simulink model "fft_test"  (Simulink 7.4)
settings: Solver=VariableStepDiscrete  StartTime=0.0  StopTime=500  RelTol=1e-3
libraries: xbsIndex_r4 x1178, casper_library_misc x68, casper_library_delays x13, casper_library_reorder x4, casper_library_ffts_twiddle x2
(part 1 of 11)
settings Model: Creator=User  LastModifiedBy=wjm
settings OptimizationCC: InitFltsAndDblsToZero=on
settings DebuggingCC: SaveWithDisabledLinksMsg=none  SaveWithParameterizedLinksMsg=none

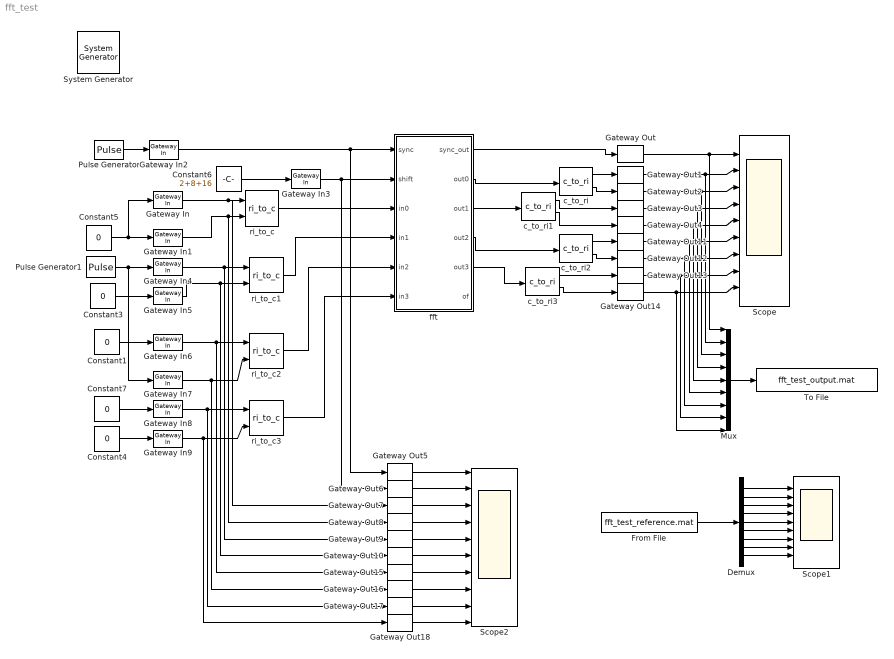
== system fft_test ==
  " System Generator" : xbsIndex_r4/ System Generator  Tag=genX  SystemSampleTime=-1  xilinxfamily=virtex5  part=xc5vsx95t  speed=-1  package=ff1136  synthesis_tool=XST  clock_wrapper=Clock Enables  directory=./netlist  testbench=off  simulink_period=1  sysclk_period=100  dcm_input_clock_period=100  incr_netlist=off  trim_vbits=Everywhere in SubSystem  dbl_ovrd=According to Block Masks  core_generation=According to Block Masks  run_coregen=off  deprecated_control=off  eval_field=0  block_type=sysgen
      settings: block_version=10.1.1
  Constant{1,3..5,7} (5 alike) : Constant  Value=0  OutDataType=sfix(16)  OutScaling=2^0
  Constant6 : Constant  Value=2+8+16  OutDataType=sfix(16)  OutScaling=2^0
  Demux : Demux  Outputs=9
  From File : FromFile  FileName=fft_test_reference.mat  SampleTime=1
  Gateway In{,1,4..9} (8 alike) : xbsIndex_r4/Gateway In  arith_type="Signed  (2's comp)"  n_bits=8  bin_pt=7  quantization=Truncate  overflow=Wrap  period=1  dbl_ovrd=off  timing_constraint=None  locs_specified=off  LOCs={}  hdl_port=on  block_type=gatewayin
      settings: infoedit="Gateway in block.  Converts inputs of type Simulink integer, double and fixed point to  Xilinx fixed point type.<P><P>Hardware notes:  In hardware these blocks become top level input ports."  block_version=10.1.1
  Gateway In2 : xbsIndex_r4/Gateway In  arith_type=Boolean  n_bits=18  bin_pt=17  quantization=Truncate  overflow=Wrap  period=1  dbl_ovrd=off  timing_constraint=None  locs_specified=off  LOCs={}  hdl_port=on  block_type=gatewayin
      settings: infoedit="Gateway in block.  Converts inputs of type Simulink integer, double and fixed point to  Xilinx fixed point type.<P><P>Hardware notes:  In hardware these blocks become top level input ports."  block_version=10.1.1
  Gateway In3 : xbsIndex_r4/Gateway In  arith_type=Unsigned  n_bits=11  bin_pt=0  quantization=Truncate  overflow=Wrap  period=1  dbl_ovrd=off  timing_constraint=None  locs_specified=off  LOCs={}  hdl_port=on  block_type=gatewayin
      settings: infoedit="Gateway in block.  Converts inputs of type Simulink integer, double and fixed point to  Xilinx fixed point type.<P><P>Hardware notes:  In hardware these blocks become top level input ports."  block_version=10.1.1
  Gateway Out{,1..18} (19 alike) : xbsIndex_r4/Gateway Out  hdl_port=on  timing_constraint=None  locs_specified=off  LOCs={}  block_type=gatewayout
      settings: infoedit="Gateway out block.  Converts Xilinx fixed point inputs into ouputs of type Simulink integer, double, or fixed point.<P><P>Hardware notes:  In hardware these blocks become top level output ports or are discarded, depending on how they are configured."  block_version=10.1.1
  Mux : Mux  Inputs=9
  Pulse Generator : DiscretePulseGenerator  Amplitude=1  Period=2^7  PulseWidth=1  PhaseDelay=11  SampleTime=1
  Pulse Generator1 : DiscretePulseGenerator  Amplitude=0.5  Period=2^4  PulseWidth=1  PhaseDelay=12  SampleTime=1
  Scope : Scope  NumInputPorts=9
      settings: YMin=-1~0~0~-5~-5~-5~-5~-5~-5  YMax=2~1~1~5~5~5~5~5~5
  Scope1 : Scope  NumInputPorts=9
      settings: YMin=-1~0~0~-5~-5~-5~-5~-5~-5  YMax=2~1~1~5~5~5~5~5~5
  Scope2 : Scope  NumInputPorts=10
      settings: YMin=-1~0~0~-5~-5~-5~-5~-5~-5~-5  YMax=2~1~1~5~5~5~5~5~5~5  SaveName=ScopeData2
  To File : ToFile  Filename=fft_test_output.mat  MatrixName=output
  c_to_ri{,1..3} (4 alike) : casper_library_misc/c_to_ri  SystemSampleTime=-1  n_bits=8  bin_pt=7
      settings: AttributesFormatString=8_7 r/i
  fft : Subsystem  AncestorBlock=casper_library_ffts/fft  mask(fft){FFTSize=6, input_bit_width=8, coeff_bit_width=8, n_inputs=2, quantization=Round  (unbiased: +/- Inf), overflow=Saturate, add_latency=2, mult_latency=3, bram_latency=1, conv_latency=2, arch=Virtex5, opt_target=multipliers, coeffs_bit_limit=8, delays_bit_limit=9, specify_mult=on, mult_spec=getfield( getfield( get_param( gcb,'UserData' ), 'parameters'),'mult_spec'), dsp48_adders=on}
      mask prompts: FFTSize "Size of FFT: (2^?)"; input_bit_width "Input/Output Bit Width"; coeff_bit_width "Coefficient Bit Width"; n_inputs "Number of Simultaneous Inputs: (2^?)"; quantization "Quantization Behavior"; overflow "Overflow Behavior"; add_latency "Add Latency"; mult_latency "Mult Latency"; bram_latency "BRAM Latency"; conv_latency "Convert latency"; arch "Architecture"; opt_target "Use less"; coeffs_bit_limit "Number bits above which to store stage's coefficients in BRAM (2^? bits)"; delays_bit_limit "Number bits above which to store stage's delays in BRAM (2^? bits)"; specify_mult "Specify multiplier use (behavioral HDL if not specified)"; mult_spec "Multiplier specification (0=core, 1=embedded, 2=behavioural) (left=1st stage)"; dsp48_adders "DSP48 adders in butterfly"
      mask init:
      | fft_init(gcb,...
      |     'FFTSize', FFTSize, ...
      |     'input_bit_width', input_bit_width, ...
      |     'coeff_bit_width', coeff_bit_width, ...
      |     'n_inputs', n_inputs, ...
      |     'quantization', quantization, ...
      |     'overflow', overflow, ...
      |     'add_latency', add_latency, ...
      |     'mult_latency', mult_latency, ...
      |     'bram_latency', bram_latency, ...
      |     'conv_latency', conv_latency, ...
      |     'arch', arch, ...
      |     'opt_target', opt_target, ...
      |     'coeffs_bit_limit', coeffs_bit_limit, ...
      |     'delays_bit_limit', delays_bit_limit, ...
      |     'specify_mult', specify_mult, ...
      |     'mult_spec', mult_spec, ...
      |     'dsp48_adders', dsp48_adders);
      settings: AttributesFormatString=|
      | 6 stages
      | (8,8)
      | Round  (unbiased: +/- Inf)
      | Saturate
      mask Help: eval('xlWeb(''http://casper.berkeley.edu/wiki/Fft'')')
      mask StyleString: edit,edit,edit,edit,popup(Truncate|Round  (unbiased: +/- Inf)|Round  (unbiased: Even Values)),popup(Wrap|Saturate|Error),edit,edit,edit,edit,popup(Virtex2Pro|Virtex5),popup(logic|multipliers),edit,edit,checkbox,edit,checkbox
      mask CallbackString:
      | % fft_size = eval(get_param(gcb, 'FFTSize'));
      | % old_vec = eval(get_param(gcb, 'mult_spec'));
      | 
      | % vec = 2.*ones(1,fft_size);
      | % old_size = length(old_vec);
      | 
      | % if(old_size <= fft_size), size = old_size;
      | % else, size = fft_size;
      | % end
      | 
      | % for n = 1:size, vec(n) = old_vec(n); end
      | % set_param(gcb, 'mult_spec', mat2str(vec));||||||||||fft_callback_arch(gcb);||||specify_mult = get_param(gcb,'specify_mult');
      | visibs = get_param(gcb, 'MaskVisibilities');
      | if( strcmp(specify_mult,'off')), visibs{16} = 'off';
      | else visibs{16} = 'on';
      | end
      | set_param(gcb, 'MaskVisibilities', visibs);
      | 
      | |% vec = eval( get_param(gcb, 'mult_spec'));
      | % vec_size = length(vec);
      | % fft_size = eval( get_param(gcb, 'FFTSize'));
      | % new_vec = 2.*ones(1, fft_size);
      | 
      | % if(vec_size <= fft_size), size = vec_size;
      | % else size = fft_size;
      | % end
      | 
      | % for n=1:size,
      | %    new_vec(n) = vec(n);
      | % end
      | % set_param(gcb, 'mult_spec', mat2str(new_vec));|fft_callback_dsp48_adders(gcb);
  ri_to_c{,1..3} (4 alike) : casper_library_misc/ri_to_c  SystemSampleTime=-1
  wires:
  Pulse Generator/1 -> Gateway In2/1
  Gateway In2/1 -> Gateway Out5/1, fft/1(sync)
  Gateway In3/1 -> Gateway Out6/1, fft/2(shift)
  fft/1(sync_out) -> Gateway Out/1
  fft/2(out0) -> c_to_ri/1
  c_to_ri/1 -> Gateway Out1/1
  c_to_ri/2 -> Gateway Out2/1
  c_to_ri1/2 -> Gateway Out4/1
  fft/3(out1) -> c_to_ri1/1
  c_to_ri1/1 -> Gateway Out3/1
  Gateway Out/1 -> Scope/1, Mux/1
  Gateway In/1 -> ri_to_c/1, Gateway Out7/1
  Gateway In1/1 -> ri_to_c/2, Gateway Out8/1
  Gateway In4/1 -> ri_to_c1/1, Gateway Out9/1
  Gateway In5/1 -> ri_to_c1/2, Gateway Out10/1
  Gateway Out1/1 -> Scope/2, Mux/2
  Gateway Out2/1 -> Scope/3, Mux/3
  Mux/1 -> To File/1
  Demux/1 -> Scope1/1
  Demux/2 -> Scope1/2
  Demux/3 -> Scope1/3
  Demux/4 -> Scope1/4
  Demux/5 -> Scope1/5
  Gateway Out5/1 -> Scope2/1
  Gateway Out6/1 -> Scope2/2
  Gateway Out7/1 -> Scope2/3
  Gateway Out8/1 -> Scope2/4
  Gateway Out9/1 -> Scope2/5
  Gateway Out10/1 -> Scope2/6
  Constant4/1 -> Gateway In9/1
  Gateway In6/1 -> ri_to_c2/1, Gateway Out15/1
  Gateway In7/1 -> ri_to_c2/2, Gateway Out16/1
  Gateway In8/1 -> ri_to_c3/1, Gateway Out17/1
  Gateway In9/1 -> ri_to_c3/2, Gateway Out18/1
  ri_to_c/1 -> fft/3(in0)
  ri_to_c1/1 -> fft/4(in1)
  ri_to_c2/1 -> fft/5(in2)
  ri_to_c3/1 -> fft/6(in3)
  c_to_ri2/1 -> Gateway Out11/1
  c_to_ri2/2 -> Gateway Out12/1
  c_to_ri3/1 -> Gateway Out13/1
  c_to_ri3/2 -> Gateway Out14/1
  Gateway Out3/1 -> Scope/4, Mux/4
  Gateway Out4/1 -> Scope/5, Mux/5
  Gateway Out11/1 -> Scope/6, Mux/6
  Gateway Out12/1 -> Scope/7, Mux/7
  Gateway Out13/1 -> Scope/8, Mux/8
  Gateway Out14/1 -> Scope/9, Mux/9
  Gateway Out15/1 -> Scope2/7
  Gateway Out16/1 -> Scope2/8
  Gateway Out17/1 -> Scope2/9
  Gateway Out18/1 -> Scope2/10
  From File/1 -> Demux/1
  Demux/6 -> Scope1/6
  Demux/7 -> Scope1/7
  Demux/8 -> Scope1/8
  Demux/9 -> Scope1/9
  Constant3/1 -> Gateway In5/1
  Constant5/1 -> Gateway In1/1, Gateway In/1
  Constant6/1 -> Gateway In3/1
  Constant1/1 -> Gateway In6/1
  Constant7/1 -> Gateway In8/1
  Pulse Generator1/1 -> Gateway In4/1, Gateway In7/1
  fft/4(out2) -> c_to_ri2/1
  fft/5(out3) -> c_to_ri3/1

== system fft_test/fft ==
  sync : Inport
  shift : Inport  Port=2
  in0 : Inport  Port=3
  in1 : Inport  Port=4
  in2 : Inport  Port=5
  in3 : Inport  Port=6
  fft_biplex0 : Subsystem  AncestorBlock=casper_library_ffts/fft_biplex  mask(fft_biplex){FFTSize=4, input_bit_width=8, coeff_bit_width=8, quantization=Round  (unbiased: +/- Inf), overflow=Saturate, add_latency=2, mult_latency=3, bram_latency=1, conv_latency=2, arch=Virtex5, opt_target=multipliers, coeffs_bit_limit=8, delays_bit_limit=9, specify_mult=on, mult_spec=getfield( getfield( get_param( gcb,'UserData' ), 'parameters'),'mult_spec'), dsp48_adders=on}
      mask prompts: FFTSize "Size of FFT: (2^? pnts)"; input_bit_width "Input/Output Bit Width"; coeff_bit_width "Coefficient Bit Width"; quantization "Quantization Behavior"; overflow "Overflow Behavior"; add_latency "Add Latency"; mult_latency "Mult Latency"; bram_latency "BRAM Latency"; conv_latency "Convert latency"; arch "Architecture"; opt_target "Use less"; coeffs_bit_limit "Number bits above which to store stage's coefficients in BRAM (2^? bits)"; delays_bit_limit "Number bits above which to implent stage's delays in BRAM (2^? bits)"; specify_mult "Specify multiplier use (behavioral HDL if not specified)"; mult_spec "Multiplier specification (0=core, 1=embedded, 2=behavioural) (left=1st stage)"; dsp48_adders "Use DSP48s for adders"
      mask init:
      | fft_biplex_init(gcb,...
      |     'FFTSize', FFTSize,...
      |     'input_bit_width', input_bit_width,...
      |     'coeff_bit_width', coeff_bit_width,...
      |     'quantization', quantization,...
      |     'overflow', overflow,...
      |     'add_latency', add_latency,...
      |     'mult_latency', mult_latency,...
      |     'bram_latency', bram_latency,...
      |     'conv_latency', conv_latency, ...
      |     'arch', arch, ...
      |     'opt_target', opt_target, ...
      |     'coeffs_bit_limit', coeffs_bit_limit, ...
      |     'delays_bit_limit', delays_bit_limit, ...
      |     'specify_mult', specify_mult,...
      |     'mult_spec', mult_spec, ...
      |     'dsp48_adders', dsp48_adders);
      settings: AttributesFormatString=|
      | 4 stages
      | Virtex5
      mask StyleString: edit,edit,edit,popup(Truncate|Round  (unbiased: +/- Inf)|Round  (unbiased: Even Values)),popup(Wrap|Saturate|Error),edit,edit,edit,edit,popup(Virtex2Pro|Virtex5),popup(logic|multipliers),edit,edit,checkbox,edit,checkbox
      mask CallbackString:
      | % fft_size = eval(get_param(gcb, 'FFTSize'));
      | % old_vec = eval(get_param(gcb, 'mult_spec'));
      | 
      | % vec = 2.*ones(1,fft_size);
      | % old_size = length(old_vec);
      | 
      | % if(old_size <= fft_size),
      | %    size = old_size;
      | % else,
      | %     size = fft_size;
      | % end
      | 
      | % for n = 1:size, vec(n) = old_vec(n); end
      | % set_param(gcb, 'mult_spec', mat2str(vec));|||||||||fft_callback_arch(gcb);||||specify_mult = get_param(gcb,'specify_mult');
      | visibs = get_param(gcb, 'MaskVisibilities');
      | 
      | if( strcmp(specify_mult,'off')), visibs{15} = 'off';
      | else, visibs{15} = 'on';
      | end
      | set_param(gcb, 'MaskVisibilities', visibs);
      | |% vec = eval( get_param(gcb, 'mult_spec'));
      | % vec_size = length(vec);
      | % fft_size = eval( get_param(gcb, 'FFTSize'));
      | % new_vec = 2.*ones(1, fft_size);
      | 
      | % if(vec_size <= fft_size), size = vec_size;
      | % else size = fft_size;
      | % end
      | 
      | % for n=1:size
      | %     new_vec(n) = vec(n);
      | % end
      | % set_param(gcb, 'mult_spec', mat2str(new_vec));|fft_callback_dsp48_adders(gcb);
  fft_biplex1 : Subsystem  AncestorBlock=casper_library_ffts/fft_biplex  mask(fft_biplex){FFTSize=4, input_bit_width=8, coeff_bit_width=8, quantization=Round  (unbiased: +/- Inf), overflow=Saturate, add_latency=2, mult_latency=3, bram_latency=1, conv_latency=2, arch=Virtex5, opt_target=multipliers, coeffs_bit_limit=8, delays_bit_limit=9, specify_mult=on, mult_spec=getfield( getfield( get_param( gcb,'UserData' ), 'parameters'),'mult_spec'), dsp48_adders=on}
      mask prompts: FFTSize "Size of FFT: (2^? pnts)"; input_bit_width "Input/Output Bit Width"; coeff_bit_width "Coefficient Bit Width"; quantization "Quantization Behavior"; overflow "Overflow Behavior"; add_latency "Add Latency"; mult_latency "Mult Latency"; bram_latency "BRAM Latency"; conv_latency "Convert latency"; arch "Architecture"; opt_target "Use less"; coeffs_bit_limit "Number bits above which to store stage's coefficients in BRAM (2^? bits)"; delays_bit_limit "Number bits above which to implent stage's delays in BRAM (2^? bits)"; specify_mult "Specify multiplier use (behavioral HDL if not specified)"; mult_spec "Multiplier specification (0=core, 1=embedded, 2=behavioural) (left=1st stage)"; dsp48_adders "Use DSP48s for adders"
      mask init: same as fft_test/fft/fft_biplex0
      settings: AttributesFormatString=|
      | 4 stages
      | Virtex5
      mask StyleString: edit,edit,edit,popup(Truncate|Round  (unbiased: +/- Inf)|Round  (unbiased: Even Values)),popup(Wrap|Saturate|Error),edit,edit,edit,edit,popup(Virtex2Pro|Virtex5),popup(logic|multipliers),edit,edit,checkbox,edit,checkbox
      mask CallbackString:
      | % fft_size = eval(get_param(gcb, 'FFTSize'));
      | % old_vec = eval(get_param(gcb, 'mult_spec'));
      | 
      | % vec = 2.*ones(1,fft_size);
      | % old_size = length(old_vec);
      | 
      | % if(old_size <= fft_size),
      | %    size = old_size;
      | % else,
      | %     size = fft_size;
      | % end
      | 
      | % for n = 1:size, vec(n) = old_vec(n); end
      | % set_param(gcb, 'mult_spec', mat2str(vec));|||||||||fft_callback_arch(gcb);||||specify_mult = get_param(gcb,'specify_mult');
      | visibs = get_param(gcb, 'MaskVisibilities');
      | 
      | if( strcmp(specify_mult,'off')), visibs{15} = 'off';
      | else, visibs{15} = 'on';
      | end
      | set_param(gcb, 'MaskVisibilities', visibs);
      | |% vec = eval( get_param(gcb, 'mult_spec'));
      | % vec_size = length(vec);
      | % fft_size = eval( get_param(gcb, 'FFTSize'));
      | % new_vec = 2.*ones(1, fft_size);
      | 
      | % if(vec_size <= fft_size), size = vec_size;
      | % else size = fft_size;
      | % end
      | 
      | % for n=1:size
      | %     new_vec(n) = vec(n);
      | % end
      | % set_param(gcb, 'mult_spec', mat2str(new_vec));|fft_callback_dsp48_adders(gcb);
  fft_direct : Subsystem  AncestorBlock=casper_library_ffts/fft_direct  mask(fft_direct){FFTSize=2, input_bit_width=8, coeff_bit_width=8, add_latency=2, mult_latency=3, bram_latency=1, conv_latency=2, quantization=Round  (unbiased: +/- Inf), overflow=Saturate, map_tail=on, LargerFFTSize=6, StartStage=5, arch=Virtex5, opt_target=multipliers, coeffs_bit_limit=8, specify_mult=on, mult_spec=[1                                      2], dsp48_adders=on}
      mask prompts: FFTSize "Size of FFT: (2^?)"; input_bit_width "Input/Output Bit Width"; coeff_bit_width "Coefficient Bit Width"; add_latency "Add Latency"; mult_latency "Mult Latency"; bram_latency "BRAM Latency"; conv_latency "Convert latency"; quantization "Quantization Behavior"; overflow "Overflow Behavior"; map_tail "Map Tail of Larger FFT"; LargerFFTSize "Size of Larger FFT (2^?):"; StartStage "Start Stage of Map Tail:"; arch "Architecture"; opt_target "Use less"; coeffs_bit_limit "Number bits above which to store stage's coefficients in BRAM (2^? bits)"; specify_mult "Specify multiplier use (behavioural HDL if not specified)"; mult_spec "Multiplier specification (0=core, 1=behavioural HDL, 2=embedded) (left=1st stage)"; dsp48_adders "DSP48 adders in butterfly"
      mask help:
      | Implements an N-point FFT with the classic
      | butterfly structure with N inputs and N outputs
      mask init:
      | fft_direct_init(gcb,...
      |     'FFTSize', FFTSize, ...
      |     'input_bit_width', input_bit_width, ...
      |     'coeff_bit_width', coeff_bit_width, ...
      |     'add_latency', add_latency, ...
      |     'mult_latency', mult_latency, ...
      |     'bram_latency', bram_latency, ...
      |     'conv_latency', conv_latency, ...
      |     'quantization', quantization, ...
      |     'overflow', overflow, ...
      |     'map_tail', map_tail, ...
      |     'LargerFFTSize', LargerFFTSize, ...
      |     'StartStage', StartStage, ...
      |     'arch', arch, ...
      |     'opt_target', opt_target, ...
      |     'coeffs_bit_limit', coeffs_bit_limit, ...
      |     'specify_mult', specify_mult, ...
      |     'mult_spec', mult_spec, ...
      |     'dsp48_adders', dsp48_adders);
      settings: AttributesFormatString=|
      | Virtex5
      | stages [5  6] of 6
      | [8,8]
      | Round  (unbiased: +/- Inf)
      | Saturate
      mask StyleString: edit,edit,edit,edit,edit,edit,edit,popup(Truncate|Round  (unbiased: +/- Inf)|Round  (unbiased: Even Values)),popup(Wrap|Saturate|Error),checkbox,edit,edit,popup(Virtex2Pro|Virtex5),popup(logic|multipliers),edit,checkbox,edit,checkbox
      mask CallbackString:
      | % fft_size = eval(get_param(gcb, 'FFTSize'));
      | % old_vec = eval(get_param(gcb, 'mult_spec'));
      | 
      | % vec = 2.*ones(1,fft_size);
      | % old_size = length(old_vec);
      | 
      | % if(old_size <= fft_size),
      | %     size = old_size;
      | % else,
      | %     size = fft_size;
      | % end
      | 
      | % for n = 1:size, vec(n) = old_vec(n); end
      | % set_param(gcb, 'mult_spec', mat2str(vec));|||||||||map_tail = get_param(gcb,'map_tail');
      | visibs = get_param(gcb, 'MaskVisibilities');
      | if( strcmp(map_tail,'off')),
      |     visibs{11} = 'off';
      |     visibs{12} = 'off';
      | else,
      |     visibs{11} = 'on';
      |     visibs{12} = 'on';
      | end
      | set_param(gcb, 'MaskVisibilities', visibs);
      | |||fft_callback_arch(gcb);|||specify_mult = get_param(gcb,'specify_mult');
      | visibs = get_param(gcb, 'MaskVisibilities');
      | if( strcmp(specify_mult,'off')), visibs{17} = 'off';
      | else, visibs{17} = 'on';
      | end
      | set_param(gcb, 'MaskVisibilities', visibs);
      | |% vec = eval( get_param(gcb, 'mult_spec'));
      | % vec_size = length(vec);
      | % fft_size = eval( get_param(gcb, 'FFTSize'));
      | % new_vec = 2.*ones(1, fft_size);
      | 
      | % if(vec_size <= fft_size), size = vec_size;
      | % else size = fft_size;
      | % end
      | 
      | % for n=1:size
      | %     new_vec(n) = vec(n);
      | % end
      | % set_param(gcb, 'mult_spec', mat2str(new_vec));|fft_callback_dsp48_adders(gcb);
  fft_unscrambler : Subsystem  AncestorBlock=casper_library_ffts/fft_unscrambler  mask(fft_unscrambler){FFTSize=6, n_inputs=2, bram_latency=1}
      mask prompts: FFTSize "Size of FFT: (2^?)"; n_inputs "Number of Simultaneous Inputs: (2^?)"; bram_latency "BRAM Latency"
      mask init:
      | fft_unscrambler_init(gcb,...
      |     'FFTSize',FFTSize,... 
      |     'n_inputs', n_inputs,...
      |     'bram_latency', bram_latency);
      settings: AttributesFormatString=FFTSize=6, n_inputs=2
  of_or : xbsIndex_r4/Logical  logical_function=OR  inputs=3  en=off  latency=1  precision=Full  arith_type=Unsigned  n_bits=16  bin_pt=0  align_bp=on  dbl_ovrd=off  block_type=logical
      settings: block_version=11.4
  slice : xbsIndex_r4/Slice  nbits=2  boolean_output=off  mode=Lower Bit Location + Width  bit1=0  base1=MSB of Input  bit0=4  base0=LSB of Input  dbl_ovrd=off  block_type=slice
  sync_out : Outport
  out0 : Outport  Port=2
  out1 : Outport  Port=3
  out2 : Outport  Port=4
  out3 : Outport  Port=5
  of : Outport  Port=6
  wires:
  in0/1 -> fft_biplex0/1(pol1)
  in1/1 -> fft_biplex0/2(pol2)
  shift/1 -> fft_biplex0/4(shift), fft_biplex1/4(shift), slice/1
  sync/1 -> fft_biplex0/3(sync), fft_biplex1/3(sync)
  fft_biplex0/3(of) -> of_or/2
  in2/1 -> fft_biplex1/1(pol1)
  in3/1 -> fft_biplex1/2(pol2)
  fft_biplex1/3(of) -> of_or/3
  slice/1 -> fft_direct/2(shift)
  fft_biplex0/4(sync_out) -> fft_direct/1(sync)
  fft_biplex0/1(pol1_out) -> fft_direct/3(in0)
  fft_biplex0/2(pol2_out) -> fft_direct/4(in1)
  fft_biplex1/1(pol1_out) -> fft_direct/5(in2)
  fft_biplex1/2(pol2_out) -> fft_direct/6(in3)
  fft_direct/6(of) -> of_or/1
  of_or/1 -> of/1
  fft_direct/1(sync_out) -> fft_unscrambler/1(sync)
  fft_unscrambler/1(sync_out) -> sync_out/1
  fft_direct/2(out0) -> fft_unscrambler/2(In1)
  fft_unscrambler/2(Out1) -> out0/1
  fft_direct/3(out1) -> fft_unscrambler/3(In2)
  fft_unscrambler/3(Out2) -> out1/1
  fft_direct/4(out2) -> fft_unscrambler/4(In3)
  fft_unscrambler/4(Out3) -> out2/1
  fft_direct/5(out3) -> fft_unscrambler/5(In4)
  fft_unscrambler/5(Out4) -> out3/1

== system fft_test/fft/fft_biplex0 ==
  pol1 : Inport  OutDataType=sfix(16)  OutScaling=2^0
  pol2 : Inport  Port=2  OutDataType=sfix(16)  OutScaling=2^0
  sync : Inport  Port=3  OutDataType=sfix(16)  OutScaling=2^0
  shift : Inport  Port=4  OutDataType=sfix(16)  OutScaling=2^0
  biplex_core : Subsystem  AncestorBlock=casper_library_ffts/biplex_core  mask(biplex_core){FFTSize=4, input_bit_width=8, coeff_bit_width=8, quantization=Round  (unbiased: +/- Inf), overflow=Saturate, add_latency=2, mult_latency=3, bram_latency=1, conv_latency=2, arch=Virtex5, opt_target=multipliers, coeffs_bit_limit=8, delays_bit_limit=9, specify_mult=on, mult_spec=getfield( getfield( get_param( gcb,'UserData' ), 'parameters'),'mult_spec'), dsp48_adders=on}
      mask prompts: FFTSize "Size of FFT: (2^? pnts)"; input_bit_width "Input/Output Bit Width"; coeff_bit_width "Coefficient Bit Width"; quantization "Quantization Behavior"; overflow "Overflow Behavior"; add_latency "Add Latency"; mult_latency "Mult Latency"; bram_latency "BRAM Latency"; conv_latency "Convert latency"; arch "Architecture"; opt_target "Use less"; coeffs_bit_limit "Number bits above which to store stage's coefficients in BRAM (2^? bits)"; delays_bit_limit "Number bits above which to implent stage's delays in BRAM (2^? bits)"; specify_mult "Specify multiplier use (behavioural HDL if not specified)"; mult_spec "Multiplier specification (0=core, 1=embedded, 2=behavioural) (left=1st stage)"; dsp48_adders "Use DSP48s for adders"
      mask init:
      | biplex_core_init(gcb,...
      |     'FFTSize', FFTSize,...
      |     'input_bit_width', input_bit_width,...
      |     'coeff_bit_width', coeff_bit_width,...
      |     'quantization', quantization,...
      |     'overflow', overflow,...
      |     'add_latency', add_latency,...
      |     'mult_latency', mult_latency,...
      |     'bram_latency', bram_latency,...
      |     'conv_latency', conv_latency, ...
      |     'arch', arch, ...
      |     'opt_target', opt_target, ...
      |     'coeffs_bit_limit', coeffs_bit_limit, ...
      |     'delays_bit_limit', delays_bit_limit, ...
      |     'specify_mult', specify_mult, ...
      |     'mult_spec', mult_spec, ...
      |     'dsp48_adders', dsp48_adders );
      settings: AttributesFormatString=|
      | 4 stages
      | reduce multipliers
      | Virtex5
      mask StyleString: edit,edit,edit,popup(Truncate|Round  (unbiased: +/- Inf)|Round  (unbiased: Even Values)),popup(Wrap|Saturate|Error),edit,edit,edit,edit,popup(Virtex2Pro|Virtex5),popup(logic|multipliers),edit,edit,checkbox,edit,checkbox
      mask CallbackString:
      | % fft_size = eval(get_param(gcb, 'FFTSize'));
      | % old_vec = eval(get_param(gcb, 'mult_spec'));
      | 
      | % vec = 2.*ones(1,fft_size);
      | % old_size = length(old_vec);
      | 
      | % if(old_size <= fft_size),
      | %    size = old_size;
      | % else,
      | %     size = fft_size;
      | % end
      | 
      | % for n = 1:size, vec(n) = old_vec(n); end
      | % set_param(gcb, 'mult_spec', mat2str(vec));|||||||||fft_callback_arch(gcb);||||specify_mult = get_param(gcb,'specify_mult');
      | visibs = get_param(gcb,'MaskVisibilities');
      | if( strcmp(specify_mult,'off')), visibs{15} = 'off';
      | else, visibs{15} = 'on';
      | end
      | set_param(gcb, 'MaskVisibilities', visibs);
      | enables = get_param(gcb,'MaskVisibilities');
      | enables{15} = 'on';
      | set_param(gcb, 'MaskEnables', enables);
      | |% vec = eval( get_param(gcb, 'mult_spec'));
      | % vec_size = length(vec);
      | % fft_size = eval( get_param(gcb, 'FFTSize'));
      | % new_vec = 2.*ones(1, fft_size);
      | 
      | % if(vec_size <= fft_size), size = vec_size;
      | % else size = fft_size;
      | % end
      | 
      | % for n=1:size
      | %     new_vec(n) = vec(n);
      | % end
      | % set_param(gcb, 'mult_spec', mat2str(new_vec));|fft_callback_dsp48_adders(gcb);
  biplex_cplx_unscrambler : Subsystem  mask{FFTSize=4, bram_latency=1}
      mask prompts: FFTSize "Size of FFT: (2^? pnts)"; bram_latency "BRAM Latency"
      mask init:
      | blk = gcb;
      | if same_state(blk, 'FFTSize', FFTSize, 'bram_latency', bram_latency), return, end
      | map = bit_reverse(0:2^(FFTSize-1)-1, FFTSize-1);
      | set_param([blk,'/reorder'],'map',mat2str([map,map+2^(FFTSize-1)]));
      | set_param([blk,'/reorder'],'bram_latency', num2str(bram_latency));
      | set_param([blk,'/reorder1'],'map',mat2str([map+2^(FFTSize-1),map]));
      | set_param([blk,'/reorder1'],'bram_latency', num2str(bram_latency));
      | save_state(blk, 'FFTSize', FFTSize, 'bram_latency', bram_latency);
  pol1_out : Outport  OutDataType=sfix(16)  OutScaling=2^0
  pol2_out : Outport  Port=2  OutDataType=sfix(16)  OutScaling=2^0
  of : Outport  Port=3  OutDataType=sfix(16)  OutScaling=2^0
  sync_out : Outport  Port=4  OutDataType=sfix(16)  OutScaling=2^0
  wires:
  biplex_core/3(of) -> of/1
  biplex_cplx_unscrambler/1(pol1) -> pol1_out/1
  shift/1 -> biplex_core/4(shift)
  sync/1 -> biplex_core/3(sync)
  pol2/1 -> biplex_core/2(pol2)
  pol1/1 -> biplex_core/1(pol1)
  biplex_core/1(out1) -> biplex_cplx_unscrambler/1(even)
  biplex_core/2(out2) -> biplex_cplx_unscrambler/2(odd)
  biplex_core/4(sync_out) -> biplex_cplx_unscrambler/3(sync)
  biplex_cplx_unscrambler/2(pol2) -> pol2_out/1
  biplex_cplx_unscrambler/3(sync_out) -> sync_out/1

== system fft_test/fft/fft_biplex1 ==
  pol1 : Inport  OutDataType=sfix(16)  OutScaling=2^0
  pol2 : Inport  Port=2  OutDataType=sfix(16)  OutScaling=2^0
  sync : Inport  Port=3  OutDataType=sfix(16)  OutScaling=2^0
  shift : Inport  Port=4  OutDataType=sfix(16)  OutScaling=2^0
  biplex_core : Subsystem  AncestorBlock=casper_library_ffts/biplex_core  mask(biplex_core){FFTSize=4, input_bit_width=8, coeff_bit_width=8, quantization=Round  (unbiased: +/- Inf), overflow=Saturate, add_latency=2, mult_latency=3, bram_latency=1, conv_latency=2, arch=Virtex5, opt_target=multipliers, coeffs_bit_limit=8, delays_bit_limit=9, specify_mult=on, mult_spec=getfield( getfield( get_param( gcb,'UserData' ), 'parameters'),'mult_spec'), dsp48_adders=on}
      mask prompts: FFTSize "Size of FFT: (2^? pnts)"; input_bit_width "Input/Output Bit Width"; coeff_bit_width "Coefficient Bit Width"; quantization "Quantization Behavior"; overflow "Overflow Behavior"; add_latency "Add Latency"; mult_latency "Mult Latency"; bram_latency "BRAM Latency"; conv_latency "Convert latency"; arch "Architecture"; opt_target "Use less"; coeffs_bit_limit "Number bits above which to store stage's coefficients in BRAM (2^? bits)"; delays_bit_limit "Number bits above which to implent stage's delays in BRAM (2^? bits)"; specify_mult "Specify multiplier use (behavioural HDL if not specified)"; mult_spec "Multiplier specification (0=core, 1=embedded, 2=behavioural) (left=1st stage)"; dsp48_adders "Use DSP48s for adders"
      mask init: same as fft_test/fft/fft_biplex0/biplex_core
      settings: AttributesFormatString=|
      | 4 stages
      | reduce multipliers
      | Virtex5
      mask StyleString: edit,edit,edit,popup(Truncate|Round  (unbiased: +/- Inf)|Round  (unbiased: Even Values)),popup(Wrap|Saturate|Error),edit,edit,edit,edit,popup(Virtex2Pro|Virtex5),popup(logic|multipliers),edit,edit,checkbox,edit,checkbox
      mask CallbackString:
      | % fft_size = eval(get_param(gcb, 'FFTSize'));
      | % old_vec = eval(get_param(gcb, 'mult_spec'));
      | 
      | % vec = 2.*ones(1,fft_size);
      | % old_size = length(old_vec);
      | 
      | % if(old_size <= fft_size),
      | %    size = old_size;
      | % else,
      | %     size = fft_size;
      | % end
      | 
      | % for n = 1:size, vec(n) = old_vec(n); end
      | % set_param(gcb, 'mult_spec', mat2str(vec));|||||||||fft_callback_arch(gcb);||||specify_mult = get_param(gcb,'specify_mult');
      | visibs = get_param(gcb,'MaskVisibilities');
      | if( strcmp(specify_mult,'off')), visibs{15} = 'off';
      | else, visibs{15} = 'on';
      | end
      | set_param(gcb, 'MaskVisibilities', visibs);
      | enables = get_param(gcb,'MaskVisibilities');
      | enables{15} = 'on';
      | set_param(gcb, 'MaskEnables', enables);
      | |% vec = eval( get_param(gcb, 'mult_spec'));
      | % vec_size = length(vec);
      | % fft_size = eval( get_param(gcb, 'FFTSize'));
      | % new_vec = 2.*ones(1, fft_size);
      | 
      | % if(vec_size <= fft_size), size = vec_size;
      | % else size = fft_size;
      | % end
      | 
      | % for n=1:size
      | %     new_vec(n) = vec(n);
      | % end
      | % set_param(gcb, 'mult_spec', mat2str(new_vec));|fft_callback_dsp48_adders(gcb);
  biplex_cplx_unscrambler : Subsystem  mask{FFTSize=4, bram_latency=1}
      mask prompts: FFTSize "Size of FFT: (2^? pnts)"; bram_latency "BRAM Latency"
      mask init: same as fft_test/fft/fft_biplex0/biplex_cplx_unscrambler
  pol1_out : Outport  OutDataType=sfix(16)  OutScaling=2^0
  pol2_out : Outport  Port=2  OutDataType=sfix(16)  OutScaling=2^0
  of : Outport  Port=3  OutDataType=sfix(16)  OutScaling=2^0
  sync_out : Outport  Port=4  OutDataType=sfix(16)  OutScaling=2^0
  wires:
  biplex_core/3(of) -> of/1
  biplex_cplx_unscrambler/1(pol1) -> pol1_out/1
  shift/1 -> biplex_core/4(shift)
  sync/1 -> biplex_core/3(sync)
  pol2/1 -> biplex_core/2(pol2)
  pol1/1 -> biplex_core/1(pol1)
  biplex_core/1(out1) -> biplex_cplx_unscrambler/1(even)
  biplex_core/2(out2) -> biplex_cplx_unscrambler/2(odd)
  biplex_core/4(sync_out) -> biplex_cplx_unscrambler/3(sync)
  biplex_cplx_unscrambler/2(pol2) -> pol2_out/1
  biplex_cplx_unscrambler/3(sync_out) -> sync_out/1

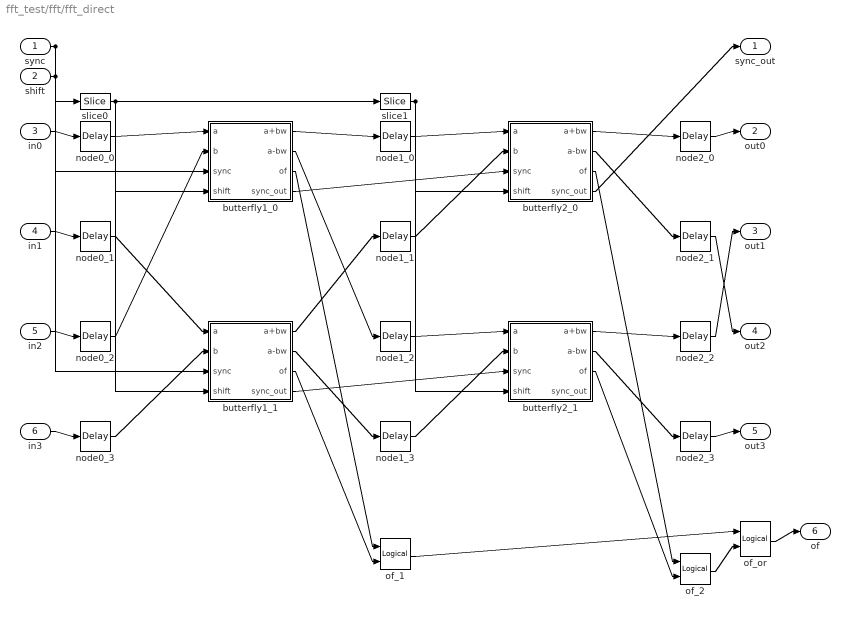
== system fft_test/fft/fft_direct ==
  sync : Inport
  shift : Inport  Port=2
  in0 : Inport  Port=3
  in1 : Inport  Port=4
  in2 : Inport  Port=5
  in3 : Inport  Port=6
  butterfly1_0 : Subsystem  AncestorBlock=casper_library_ffts/butterfly_direct  mask(butterfly_direct){biplex=off, FFTSize=6, Coeffs=getfield( getfield( get_param( gcb,'UserData' ), 'parameters'),'Coeffs'), StepPeriod=0, coeffs_bram=off, coeff_bit_width=8, input_bit_width=8, bram_latency=1, add_latency=2, mult_latency=3, conv_latency=2, quantization=Round  (unbiased: +/- Inf), overflow=Saturate, arch=Virtex5, opt_target=multipliers, use_hdl=off, use_embedded=on, dsp48_adders=on}
      mask prompts: biplex "Used in biplex FFT"; FFTSize "Size of FFT: (2^?)"; Coeffs "Coefficients: (0 to 2^(FFTSize-1)-1)"; StepPeriod "Coefficient Step Period: (2^?)"; coeffs_bram "Implement coefficients in BRAM"; coeff_bit_width "Coefficient Bit Width"; input_bit_width "Input/Output Bit Width:"; bram_latency "BRAM Latency"; add_latency "Add Latency"; mult_latency "Mult Latency"; conv_latency "Convert latency"; quantization "Quantization Behavior"; overflow "Overflow Behavior"; arch "Architecture"; opt_target "Use less"; use_hdl "Use behavioural HDL for multipliers"; use_embedded "Use embedded multipliers"; dsp48_adders "Use DSP48s for adders"
      mask init:
      | butterfly_direct_init(gcb,...
      |     'biplex', biplex,...
      |     'FFTSize', FFTSize,...
      |     'Coeffs', Coeffs,...
      |     'coeff_bit_width', coeff_bit_width,...
      |     'StepPeriod', StepPeriod,...
      |     'input_bit_width', input_bit_width,...
      |     'add_latency', add_latency,...
      |     'mult_latency', mult_latency,...
      |     'bram_latency', bram_latency,...
      |     'conv_latency', conv_latency, ...
      |     'coeffs_bram', coeffs_bram,...    
      |     'quantization', quantization,...
      |     'overflow', overflow,...
      |     'arch', arch,...
      |     'opt_target', opt_target,...
      |     'use_hdl', use_hdl,...
      |     'use_embedded', use_embedded,...
      |     'dsp48_adders', dsp48_adders);
      settings: AttributesFormatString=|
      | twiddle_general_3mult
      | coeffs in slices
      mask StyleString: checkbox,edit,edit,edit,checkbox,edit,edit,edit,edit,edit,edit,popup(Truncate|Round  (unbiased: +/- Inf)|Round  (unbiased: Even Values)),popup(Wrap|Saturate|Error),popup(Virtex2Pro|Virtex5),popup(logic|multipliers),checkbox,checkbox,checkbox
      mask CallbackString:
      | ||%coeffs = eval(get_param(gcb,'Coeffs'));
      | %visibs = get_param(gcb,'MaskVisibilities');
      | %if length(coeffs) == 1,
      | %    visibs{4} = 'off'; visibs{5} = 'off';
      | %    visibs{6} = 'off';
      | %else
      | %    visibs{4} = 'on';
      | %    visibs{5} = 'on'; visibs{6} = 'on';
      | %end
      | %set_param(gcb, 'MaskVisibilities', visibs);|%coeffs = eval(get_param(gcb,'Coeffs'));
      | %visibs = get_param(gcb,'MaskVisibilities');
      | %if length(coeffs) == 1,
      | %    visibs{4} = 'off'; visibs{5} = 'off';
      | %    visibs{6} = 'off';
      | %else
      | %%    visibs{4} = 'on';
      | %    visibs{5} = 'on'; visibs{6} = 'on';
      | %end
      | %set_param(gcb, 'MaskVisibilities', visibs);|%coeffs = eval(get_param(gcb,'Coeffs'));
      | %visibs = get_param(gcb,'MaskVisibilities');
      | %if length(coeffs) == 1,
      | %    visibs{5} = 'off'; visibs{6} = 'off';
      | %    visibs{7} = 'off';
      | %else
      | %    visibs{5} = 'on';
      | %    visibs{6} = 'on'; visibs{7} = 'on';
      | %end
      | %set_param(gcb, 'MaskVisibilities', visibs);|||||||||fft_callback_arch(gcb);||use_hdl = get_param(gcb,'use_hdl');
      | visibs = get_param(gcb, 'MaskVisibilities');
      | if( strcmp(use_hdl,'on')),
      |     set_param(gcb, 'use_embedded','off');
      |     visibs{17} = 'off';
      | else,
      |     visibs{17} = 'on';
      | end
      |     set_param(gcb, 'MaskVisibilities',visibs);||fft_callback_dsp48_adders(gcb);
  butterfly1_1 : Subsystem  AncestorBlock=casper_library_ffts/butterfly_direct  mask(butterfly_direct){biplex=off, FFTSize=6, Coeffs=getfield( getfield( get_param( gcb,'UserData' ), 'parameters'),'Coeffs'), StepPeriod=0, coeffs_bram=off, coeff_bit_width=8, input_bit_width=8, bram_latency=1, add_latency=2, mult_latency=3, conv_latency=2, quantization=Round  (unbiased: +/- Inf), overflow=Saturate, arch=Virtex5, opt_target=multipliers, use_hdl=off, use_embedded=on, dsp48_adders=on}
      mask prompts: biplex "Used in biplex FFT"; FFTSize "Size of FFT: (2^?)"; Coeffs "Coefficients: (0 to 2^(FFTSize-1)-1)"; StepPeriod "Coefficient Step Period: (2^?)"; coeffs_bram "Implement coefficients in BRAM"; coeff_bit_width "Coefficient Bit Width"; input_bit_width "Input/Output Bit Width:"; bram_latency "BRAM Latency"; add_latency "Add Latency"; mult_latency "Mult Latency"; conv_latency "Convert latency"; quantization "Quantization Behavior"; overflow "Overflow Behavior"; arch "Architecture"; opt_target "Use less"; use_hdl "Use behavioural HDL for multipliers"; use_embedded "Use embedded multipliers"; dsp48_adders "Use DSP48s for adders"
      mask init: same as fft_test/fft/fft_direct/butterfly1_0
      settings: AttributesFormatString=|
      | twiddle_general_3mult
      | coeffs in slices
      mask StyleString: checkbox,edit,edit,edit,checkbox,edit,edit,edit,edit,edit,edit,popup(Truncate|Round  (unbiased: +/- Inf)|Round  (unbiased: Even Values)),popup(Wrap|Saturate|Error),popup(Virtex2Pro|Virtex5),popup(logic|multipliers),checkbox,checkbox,checkbox
      mask CallbackString:
      | ||%coeffs = eval(get_param(gcb,'Coeffs'));
      | %visibs = get_param(gcb,'MaskVisibilities');
      | %if length(coeffs) == 1,
      | %    visibs{4} = 'off'; visibs{5} = 'off';
      | %    visibs{6} = 'off';
      | %else
      | %    visibs{4} = 'on';
      | %    visibs{5} = 'on'; visibs{6} = 'on';
      | %end
      | %set_param(gcb, 'MaskVisibilities', visibs);|%coeffs = eval(get_param(gcb,'Coeffs'));
      | %visibs = get_param(gcb,'MaskVisibilities');
      | %if length(coeffs) == 1,
      | %    visibs{4} = 'off'; visibs{5} = 'off';
      | %    visibs{6} = 'off';
      | %else
      | %%    visibs{4} = 'on';
      | %    visibs{5} = 'on'; visibs{6} = 'on';
      | %end
      | %set_param(gcb, 'MaskVisibilities', visibs);|%coeffs = eval(get_param(gcb,'Coeffs'));
      | %visibs = get_param(gcb,'MaskVisibilities');
      | %if length(coeffs) == 1,
      | %    visibs{5} = 'off'; visibs{6} = 'off';
      | %    visibs{7} = 'off';
      | %else
      | %    visibs{5} = 'on';
      | %    visibs{6} = 'on'; visibs{7} = 'on';
      | %end
      | %set_param(gcb, 'MaskVisibilities', visibs);|||||||||fft_callback_arch(gcb);||use_hdl = get_param(gcb,'use_hdl');
      | visibs = get_param(gcb, 'MaskVisibilities');
      | if( strcmp(use_hdl,'on')),
      |     set_param(gcb, 'use_embedded','off');
      |     visibs{17} = 'off';
      | else,
      |     visibs{17} = 'on';
      | end
      |     set_param(gcb, 'MaskVisibilities',visibs);||fft_callback_dsp48_adders(gcb);
  butterfly2_0 : Subsystem  AncestorBlock=casper_library_ffts/butterfly_direct  mask(butterfly_direct){biplex=off, FFTSize=6, Coeffs=getfield( getfield( get_param( gcb,'UserData' ), 'parameters'),'Coeffs'), StepPeriod=0, coeffs_bram=off, coeff_bit_width=8, input_bit_width=8, bram_latency=1, add_latency=2, mult_latency=3, conv_latency=2, quantization=Round  (unbiased: +/- Inf), overflow=Saturate, arch=Virtex5, opt_target=multipliers, use_hdl=on, use_embedded=off, dsp48_adders=on}
      mask prompts: biplex "Used in biplex FFT"; FFTSize "Size of FFT: (2^?)"; Coeffs "Coefficients: (0 to 2^(FFTSize-1)-1)"; StepPeriod "Coefficient Step Period: (2^?)"; coeffs_bram "Implement coefficients in BRAM"; coeff_bit_width "Coefficient Bit Width"; input_bit_width "Input/Output Bit Width:"; bram_latency "BRAM Latency"; add_latency "Add Latency"; mult_latency "Mult Latency"; conv_latency "Convert latency"; quantization "Quantization Behavior"; overflow "Overflow Behavior"; arch "Architecture"; opt_target "Use less"; use_hdl "Use behavioural HDL for multipliers"; use_embedded "Use embedded multipliers"; dsp48_adders "Use DSP48s for adders"
      mask init: same as fft_test/fft/fft_direct/butterfly1_0
      settings: AttributesFormatString=|
      | twiddle_general_3mult
      | coeffs in slices
      mask StyleString: checkbox,edit,edit,edit,checkbox,edit,edit,edit,edit,edit,edit,popup(Truncate|Round  (unbiased: +/- Inf)|Round  (unbiased: Even Values)),popup(Wrap|Saturate|Error),popup(Virtex2Pro|Virtex5),popup(logic|multipliers),checkbox,checkbox,checkbox
      mask CallbackString:
      | ||%coeffs = eval(get_param(gcb,'Coeffs'));
      | %visibs = get_param(gcb,'MaskVisibilities');
      | %if length(coeffs) == 1,
      | %    visibs{4} = 'off'; visibs{5} = 'off';
      | %    visibs{6} = 'off';
      | %else
      | %    visibs{4} = 'on';
      | %    visibs{5} = 'on'; visibs{6} = 'on';
      | %end
      | %set_param(gcb, 'MaskVisibilities', visibs);|%coeffs = eval(get_param(gcb,'Coeffs'));
      | %visibs = get_param(gcb,'MaskVisibilities');
      | %if length(coeffs) == 1,
      | %    visibs{4} = 'off'; visibs{5} = 'off';
      | %    visibs{6} = 'off';
      | %else
      | %%    visibs{4} = 'on';
      | %    visibs{5} = 'on'; visibs{6} = 'on';
      | %end
      | %set_param(gcb, 'MaskVisibilities', visibs);|%coeffs = eval(get_param(gcb,'Coeffs'));
      | %visibs = get_param(gcb,'MaskVisibilities');
      | %if length(coeffs) == 1,
      | %    visibs{5} = 'off'; visibs{6} = 'off';
      | %    visibs{7} = 'off';
      | %else
      | %    visibs{5} = 'on';
      | %    visibs{6} = 'on'; visibs{7} = 'on';
      | %end
      | %set_param(gcb, 'MaskVisibilities', visibs);|||||||||fft_callback_arch(gcb);||use_hdl = get_param(gcb,'use_hdl');
      | visibs = get_param(gcb, 'MaskVisibilities');
      | if( strcmp(use_hdl,'on')),
      |     set_param(gcb, 'use_embedded','off');
      |     visibs{17} = 'off';
      | else,
      |     visibs{17} = 'on';
      | end
      |     set_param(gcb, 'MaskVisibilities',visibs);||fft_callback_dsp48_adders(gcb);
  butterfly2_1 : Subsystem  AncestorBlock=casper_library_ffts/butterfly_direct  mask(butterfly_direct){biplex=off, FFTSize=6, Coeffs=getfield( getfield( get_param( gcb,'UserData' ), 'parameters'),'Coeffs'), StepPeriod=0, coeffs_bram=off, coeff_bit_width=8, input_bit_width=8, bram_latency=1, add_latency=2, mult_latency=3, conv_latency=2, quantization=Round  (unbiased: +/- Inf), overflow=Saturate, arch=Virtex5, opt_target=multipliers, use_hdl=on, use_embedded=off, dsp48_adders=on}
      mask prompts: biplex "Used in biplex FFT"; FFTSize "Size of FFT: (2^?)"; Coeffs "Coefficients: (0 to 2^(FFTSize-1)-1)"; StepPeriod "Coefficient Step Period: (2^?)"; coeffs_bram "Implement coefficients in BRAM"; coeff_bit_width "Coefficient Bit Width"; input_bit_width "Input/Output Bit Width:"; bram_latency "BRAM Latency"; add_latency "Add Latency"; mult_latency "Mult Latency"; conv_latency "Convert latency"; quantization "Quantization Behavior"; overflow "Overflow Behavior"; arch "Architecture"; opt_target "Use less"; use_hdl "Use behavioural HDL for multipliers"; use_embedded "Use embedded multipliers"; dsp48_adders "Use DSP48s for adders"
      mask init: same as fft_test/fft/fft_direct/butterfly1_0
      settings: AttributesFormatString=|
      | twiddle_general_3mult
      | coeffs in slices
      mask StyleString: checkbox,edit,edit,edit,checkbox,edit,edit,edit,edit,edit,edit,popup(Truncate|Round  (unbiased: +/- Inf)|Round  (unbiased: Even Values)),popup(Wrap|Saturate|Error),popup(Virtex2Pro|Virtex5),popup(logic|multipliers),checkbox,checkbox,checkbox
      mask CallbackString:
      | ||%coeffs = eval(get_param(gcb,'Coeffs'));
      | %visibs = get_param(gcb,'MaskVisibilities');
      | %if length(coeffs) == 1,
      | %    visibs{4} = 'off'; visibs{5} = 'off';
      | %    visibs{6} = 'off';
      | %else
      | %    visibs{4} = 'on';
      | %    visibs{5} = 'on'; visibs{6} = 'on';
      | %end
      | %set_param(gcb, 'MaskVisibilities', visibs);|%coeffs = eval(get_param(gcb,'Coeffs'));
      | %visibs = get_param(gcb,'MaskVisibilities');
      | %if length(coeffs) == 1,
      | %    visibs{4} = 'off'; visibs{5} = 'off';
      | %    visibs{6} = 'off';
      | %else
      | %%    visibs{4} = 'on';
      | %    visibs{5} = 'on'; visibs{6} = 'on';
      | %end
      | %set_param(gcb, 'MaskVisibilities', visibs);|%coeffs = eval(get_param(gcb,'Coeffs'));
      | %visibs = get_param(gcb,'MaskVisibilities');
      | %if length(coeffs) == 1,
      | %    visibs{5} = 'off'; visibs{6} = 'off';
      | %    visibs{7} = 'off';
      | %else
      | %    visibs{5} = 'on';
      | %    visibs{6} = 'on'; visibs{7} = 'on';
      | %end
      | %set_param(gcb, 'MaskVisibilities', visibs);|||||||||fft_callback_arch(gcb);||use_hdl = get_param(gcb,'use_hdl');
      | visibs = get_param(gcb, 'MaskVisibilities');
      | if( strcmp(use_hdl,'on')),
      |     set_param(gcb, 'use_embedded','off');
      |     visibs{17} = 'off';
      | else,
      |     visibs{17} = 'on';
      | end
      |     set_param(gcb, 'MaskVisibilities',visibs);||fft_callback_dsp48_adders(gcb);
  node0_{0..3} (4 alike) : xbsIndex_r4/Delay  en=off  latency=0  dbl_ovrd=off  reg_retiming=off  block_type=delay
      settings: block_version=11.4
  node1_{0..3} (4 alike) : xbsIndex_r4/Delay  en=off  latency=0  dbl_ovrd=off  reg_retiming=off  block_type=delay
      settings: block_version=11.4
  node2_{0..3} (4 alike) : xbsIndex_r4/Delay  en=off  latency=0  dbl_ovrd=off  reg_retiming=off  block_type=delay
      settings: block_version=11.4
  of_1 : xbsIndex_r4/Logical  logical_function=OR  inputs=2  en=off  latency=1  precision=Full  arith_type=Unsigned  n_bits=16  bin_pt=0  align_bp=on  dbl_ovrd=off  block_type=logical
      settings: block_version=11.4
  of_2 : xbsIndex_r4/Logical  logical_function=OR  inputs=2  en=off  latency=1  precision=Full  arith_type=Unsigned  n_bits=16  bin_pt=0  align_bp=on  dbl_ovrd=off  block_type=logical
      settings: block_version=11.4
  of_or : xbsIndex_r4/Logical  logical_function=OR  inputs=2  en=off  latency=0  precision=Full  arith_type=Unsigned  n_bits=16  bin_pt=0  align_bp=on  dbl_ovrd=off  block_type=logical
      settings: block_version=11.4
  slice0 : xbsIndex_r4/Slice  nbits=1  boolean_output=on  mode=Lower Bit Location + Width  bit1=0  base1=MSB of Input  bit0=0  base0=LSB of Input  dbl_ovrd=off  block_type=slice
  slice1 : xbsIndex_r4/Slice  nbits=1  boolean_output=on  mode=Lower Bit Location + Width  bit1=0  base1=MSB of Input  bit0=1  base0=LSB of Input  dbl_ovrd=off  block_type=slice
  sync_out : Outport
  out0 : Outport  Port=2
  out1 : Outport  Port=3
  out2 : Outport  Port=4
  out3 : Outport  Port=5
  of : Outport  Port=6
  wires:
  of_or/1 -> of/1
  in0/1 -> node0_0/1
  in1/1 -> node0_1/1
  in2/1 -> node0_2/1
  in3/1 -> node0_3/1
  shift/1 -> slice0/1, slice1/1
  node2_0/1 -> out0/1
  node2_1/1 -> out2/1
  node2_2/1 -> out1/1
  node2_3/1 -> out3/1
  of_1/1 -> of_or/1
  node0_0/1 -> butterfly1_0/1(a)
  node0_2/1 -> butterfly1_0/2(b)
  butterfly1_0/1(a+bw) -> node1_0/1
  butterfly1_0/2(a-bw) -> node1_2/1
  sync/1 -> butterfly1_0/3(sync), butterfly1_1/3(sync)
  slice0/1 -> butterfly1_0/4(shift), butterfly1_1/4(shift)
  butterfly1_0/3(of) -> of_1/1
  node0_1/1 -> butterfly1_1/1(a)
  node0_3/1 -> butterfly1_1/2(b)
  butterfly1_1/1(a+bw) -> node1_1/1
  butterfly1_1/2(a-bw) -> node1_3/1
  butterfly1_1/3(of) -> of_1/2
  of_2/1 -> of_or/2
  node1_0/1 -> butterfly2_0/1(a)
  node1_1/1 -> butterfly2_0/2(b)
  butterfly2_0/1(a+bw) -> node2_0/1
  butterfly2_0/2(a-bw) -> node2_1/1
  butterfly1_0/4(sync_out) -> butterfly2_0/3(sync)
  butterfly2_0/4(sync_out) -> sync_out/1
  slice1/1 -> butterfly2_0/4(shift), butterfly2_1/4(shift)
  butterfly2_0/3(of) -> of_2/1
  node1_2/1 -> butterfly2_1/1(a)
  node1_3/1 -> butterfly2_1/2(b)
  butterfly2_1/1(a+bw) -> node2_2/1
  butterfly2_1/2(a-bw) -> node2_3/1
  butterfly1_1/4(sync_out) -> butterfly2_1/3(sync)
  butterfly2_1/3(of) -> of_2/2
